simulink model "tp_thyr_rect_sm"  (R2026a)
settings: Solver=daessc  StopTime=simlength  FixedStep=Ts  MaxStep=Ts  RelTol=Ts  AbsTol=Ts  EnableMultiTasking=on
values from neighbouring files (symbols this model uses):
  I_FS = Iout_dc_nom * margin_factor    (= 103.5)    [init_model.m]
  kgrid = 1    [init_model.m]
  LFu_dc = 1.2e-3    (= 0.0012)    [init_model.m]
  pll_i1 = 80    [init_model.m]
  pll_p = 1    [init_model.m]
  RLFu_dc = 2e-4    (= 0.0002)    [init_model.m]
  Rload = 1.2/4    (= 0.3)    [init_model.m]
  Tc = 1e-5    (= 1e-05)    [init_model.m]
  Tcontrol_rect = tPWM_RECT    (= 0.0002)    [init_model.m]
  Ts = Tc/1    (= 1e-05)    [init_model.m]
  V_FS = Vout_dc_nom * margin_factor    (= 391)    [init_model.m]
  Vnom_ac_adc = 400/sqrt(3)*sqrt(2)    [init_model.m]
  Vphase1 = Vline1/sqrt(3)    [init_model.m]
  w_grid = f_grid*2*pi    (= 314.159265359)    [init_model.m]
undefined symbols (not defined in the file or in its folder): magnitude
libraries: fl_lib x248, nesl_utility x39, ee_lib x28
(part 5 of 5)

== system tp_thyr_rect_sm/Line/BR1/firing4/oscillator ==
  Data Type Conversion : DataTypeConversion  OutDataTypeStr=double  SaturateOnIntegerOverflow=off  RndMeth=Floor
  Logical Operator1 : Logic  Operator=NOT  AllPortsSameDT=off  OutDataTypeStr=boolean
  Simulink-PS Converter : nesl_utility/Simulink-PS Converter  PhysicalDomain=network_engine_domain  SubClassName=ps_input  LeftPortType=input  RightPortType=output  PseudoPeriodic=off  Frequencies=[]  NoiseDistribution=none  NoiseParameters=[]  Unit=1  AffineConversion=off  FilteringAndDerivatives=provide  SimscapeFilterOrder=1  InputFilterTimeConstant=0.001  UdotUserProvided=0
  Unit Delay1 : UnitDelay  SampleTime=Tcontrol_rect
  output : PMIOPort  Side=Right
  wires:
  Data Type Conversion/1 -> Simulink-PS Converter/1
  Unit Delay1/1 -> Logical Operator1/1
  Logical Operator1/1 -> Unit Delay1/1, Data Type Conversion/1
  connections:
  Simulink-PS Converter/RConn1 -- output/RConn1

== system tp_thyr_rect_sm/Line/BR1/firing5/oscillator ==
  Data Type Conversion : DataTypeConversion  OutDataTypeStr=double  SaturateOnIntegerOverflow=off  RndMeth=Floor
  Logical Operator1 : Logic  Operator=NOT  AllPortsSameDT=off  OutDataTypeStr=boolean
  Simulink-PS Converter : nesl_utility/Simulink-PS Converter  PhysicalDomain=network_engine_domain  SubClassName=ps_input  LeftPortType=input  RightPortType=output  PseudoPeriodic=off  Frequencies=[]  NoiseDistribution=none  NoiseParameters=[]  Unit=1  AffineConversion=off  FilteringAndDerivatives=provide  SimscapeFilterOrder=1  InputFilterTimeConstant=0.001  UdotUserProvided=0
  Unit Delay1 : UnitDelay  SampleTime=Tcontrol_rect
  output : PMIOPort  Side=Right
  wires:
  Logical Operator1/1 -> Data Type Conversion/1, Unit Delay1/1
  Unit Delay1/1 -> Logical Operator1/1
  Data Type Conversion/1 -> Simulink-PS Converter/1
  connections:
  Simulink-PS Converter/RConn1 -- output/RConn1

== system tp_thyr_rect_sm/Line/BR1/firing6/oscillator ==
  Data Type Conversion : DataTypeConversion  OutDataTypeStr=double  SaturateOnIntegerOverflow=off  RndMeth=Floor
  Logical Operator1 : Logic  Operator=NOT  AllPortsSameDT=off  OutDataTypeStr=boolean
  Simulink-PS Converter : nesl_utility/Simulink-PS Converter  PhysicalDomain=network_engine_domain  SubClassName=ps_input  LeftPortType=input  RightPortType=output  PseudoPeriodic=off  Frequencies=[]  NoiseDistribution=none  NoiseParameters=[]  Unit=1  AffineConversion=off  FilteringAndDerivatives=provide  SimscapeFilterOrder=1  InputFilterTimeConstant=0.001  UdotUserProvided=0
  Unit Delay1 : UnitDelay  SampleTime=Tcontrol_rect
  output : PMIOPort  Side=Right
  wires:
  Data Type Conversion/1 -> Simulink-PS Converter/1
  Unit Delay1/1 -> Logical Operator1/1
  Logical Operator1/1 -> Unit Delay1/1, Data Type Conversion/1
  connections:
  Simulink-PS Converter/RConn1 -- output/RConn1

== system tp_thyr_rect_sm/Line/BR2/firing1/oscillator ==
  Data Type Conversion : DataTypeConversion  OutDataTypeStr=double  SaturateOnIntegerOverflow=off  RndMeth=Floor
  Logical Operator1 : Logic  Operator=NOT  AllPortsSameDT=off  OutDataTypeStr=boolean
  Simulink-PS Converter : nesl_utility/Simulink-PS Converter  PhysicalDomain=network_engine_domain  SubClassName=ps_input  LeftPortType=input  RightPortType=output  PseudoPeriodic=off  Frequencies=[]  NoiseDistribution=none  NoiseParameters=[]  Unit=1  AffineConversion=off  FilteringAndDerivatives=provide  SimscapeFilterOrder=1  InputFilterTimeConstant=0.001  UdotUserProvided=0
  Unit Delay1 : UnitDelay  SampleTime=Tcontrol_rect
  output : PMIOPort  Side=Right
  wires:
  Data Type Conversion/1 -> Simulink-PS Converter/1
  Unit Delay1/1 -> Logical Operator1/1
  Logical Operator1/1 -> Unit Delay1/1, Data Type Conversion/1
  connections:
  Simulink-PS Converter/RConn1 -- output/RConn1

== system tp_thyr_rect_sm/Line/BR2/firing2/oscillator ==
  Data Type Conversion : DataTypeConversion  OutDataTypeStr=double  SaturateOnIntegerOverflow=off  RndMeth=Floor
  Logical Operator1 : Logic  Operator=NOT  AllPortsSameDT=off  OutDataTypeStr=boolean
  Simulink-PS Converter : nesl_utility/Simulink-PS Converter  PhysicalDomain=network_engine_domain  SubClassName=ps_input  LeftPortType=input  RightPortType=output  PseudoPeriodic=off  Frequencies=[]  NoiseDistribution=none  NoiseParameters=[]  Unit=1  AffineConversion=off  FilteringAndDerivatives=provide  SimscapeFilterOrder=1  InputFilterTimeConstant=0.001  UdotUserProvided=0
  Unit Delay1 : UnitDelay  SampleTime=Tcontrol_rect
  output : PMIOPort  Side=Right
  wires:
  Logical Operator1/1 -> Data Type Conversion/1, Unit Delay1/1
  Unit Delay1/1 -> Logical Operator1/1
  Data Type Conversion/1 -> Simulink-PS Converter/1
  connections:
  Simulink-PS Converter/RConn1 -- output/RConn1

== system tp_thyr_rect_sm/Line/BR2/firing3/oscillator ==
  Data Type Conversion : DataTypeConversion  OutDataTypeStr=double  SaturateOnIntegerOverflow=off  RndMeth=Floor
  Logical Operator1 : Logic  Operator=NOT  AllPortsSameDT=off  OutDataTypeStr=boolean
  Simulink-PS Converter : nesl_utility/Simulink-PS Converter  PhysicalDomain=network_engine_domain  SubClassName=ps_input  LeftPortType=input  RightPortType=output  PseudoPeriodic=off  Frequencies=[]  NoiseDistribution=none  NoiseParameters=[]  Unit=1  AffineConversion=off  FilteringAndDerivatives=provide  SimscapeFilterOrder=1  InputFilterTimeConstant=0.001  UdotUserProvided=0
  Unit Delay1 : UnitDelay  SampleTime=Tcontrol_rect
  output : PMIOPort  Side=Right
  wires:
  Data Type Conversion/1 -> Simulink-PS Converter/1
  Unit Delay1/1 -> Logical Operator1/1
  Logical Operator1/1 -> Unit Delay1/1, Data Type Conversion/1
  connections:
  Simulink-PS Converter/RConn1 -- output/RConn1

== system tp_thyr_rect_sm/Line/BR2/firing4/oscillator ==
  Data Type Conversion : DataTypeConversion  OutDataTypeStr=double  SaturateOnIntegerOverflow=off  RndMeth=Floor
  Logical Operator1 : Logic  Operator=NOT  AllPortsSameDT=off  OutDataTypeStr=boolean
  Simulink-PS Converter : nesl_utility/Simulink-PS Converter  PhysicalDomain=network_engine_domain  SubClassName=ps_input  LeftPortType=input  RightPortType=output  PseudoPeriodic=off  Frequencies=[]  NoiseDistribution=none  NoiseParameters=[]  Unit=1  AffineConversion=off  FilteringAndDerivatives=provide  SimscapeFilterOrder=1  InputFilterTimeConstant=0.001  UdotUserProvided=0
  Unit Delay1 : UnitDelay  SampleTime=Tcontrol_rect
  output : PMIOPort  Side=Right
  wires:
  Logical Operator1/1 -> Data Type Conversion/1, Unit Delay1/1
  Unit Delay1/1 -> Logical Operator1/1
  Data Type Conversion/1 -> Simulink-PS Converter/1
  connections:
  Simulink-PS Converter/RConn1 -- output/RConn1

== system tp_thyr_rect_sm/Line/BR2/firing5/oscillator ==
  Data Type Conversion : DataTypeConversion  OutDataTypeStr=double  SaturateOnIntegerOverflow=off  RndMeth=Floor
  Logical Operator1 : Logic  Operator=NOT  AllPortsSameDT=off  OutDataTypeStr=boolean
  Simulink-PS Converter : nesl_utility/Simulink-PS Converter  PhysicalDomain=network_engine_domain  SubClassName=ps_input  LeftPortType=input  RightPortType=output  PseudoPeriodic=off  Frequencies=[]  NoiseDistribution=none  NoiseParameters=[]  Unit=1  AffineConversion=off  FilteringAndDerivatives=provide  SimscapeFilterOrder=1  InputFilterTimeConstant=0.001  UdotUserProvided=0
  Unit Delay1 : UnitDelay  SampleTime=Tcontrol_rect
  output : PMIOPort  Side=Right
  wires:
  Data Type Conversion/1 -> Simulink-PS Converter/1
  Unit Delay1/1 -> Logical Operator1/1
  Logical Operator1/1 -> Unit Delay1/1, Data Type Conversion/1
  connections:
  Simulink-PS Converter/RConn1 -- output/RConn1

== system tp_thyr_rect_sm/Line/BR2/firing6/oscillator ==
  Data Type Conversion : DataTypeConversion  OutDataTypeStr=double  SaturateOnIntegerOverflow=off  RndMeth=Floor
  Logical Operator1 : Logic  Operator=NOT  AllPortsSameDT=off  OutDataTypeStr=boolean
  Simulink-PS Converter : nesl_utility/Simulink-PS Converter  PhysicalDomain=network_engine_domain  SubClassName=ps_input  LeftPortType=input  RightPortType=output  PseudoPeriodic=off  Frequencies=[]  NoiseDistribution=none  NoiseParameters=[]  Unit=1  AffineConversion=off  FilteringAndDerivatives=provide  SimscapeFilterOrder=1  InputFilterTimeConstant=0.001  UdotUserProvided=0
  Unit Delay1 : UnitDelay  SampleTime=Tcontrol_rect
  output : PMIOPort  Side=Right
  wires:
  Logical Operator1/1 -> Data Type Conversion/1, Unit Delay1/1
  Unit Delay1/1 -> Logical Operator1/1
  Data Type Conversion/1 -> Simulink-PS Converter/1
  connections:
  Simulink-PS Converter/RConn1 -- output/RConn1

== system tp_thyr_rect_sm/Line/C-caller ctrl/Subsystem2/oscillator ==
  In1 : Inport
  Logical Operator1 : Logic  Operator=NOT  AllPortsSameDT=off  OutDataTypeStr=boolean
  Product : Product
  Unit Delay1 : UnitDelay  SampleTime=Tcontrol_rect
  Out1 : Outport
  wires:
  Unit Delay1/1 -> Logical Operator1/1
  Logical Operator1/1 -> Product/1, Unit Delay1/1
  Product/1 -> Out1/1
  In1/1 -> Product/2

== system tp_thyr_rect_sm/Line/C-caller ctrl/Subsystem2/oscillator1 ==
  In1 : Inport
  Logical Operator1 : Logic  Operator=NOT  AllPortsSameDT=off  OutDataTypeStr=boolean
  Product : Product
  Unit Delay1 : UnitDelay  SampleTime=Tcontrol_rect
  Out1 : Outport
  wires:
  In1/1 -> Product/2
  Product/1 -> Out1/1
  Logical Operator1/1 -> Unit Delay1/1, Product/1
  Unit Delay1/1 -> Logical Operator1/1

== system tp_thyr_rect_sm/Line/C-caller ctrl/Subsystem2/oscillator2 ==
  In1 : Inport
  Logical Operator1 : Logic  Operator=NOT  AllPortsSameDT=off  OutDataTypeStr=boolean
  Product : Product
  Unit Delay1 : UnitDelay  SampleTime=Tcontrol_rect
  Out1 : Outport
  wires:
  Unit Delay1/1 -> Logical Operator1/1
  Logical Operator1/1 -> Product/1, Unit Delay1/1
  Product/1 -> Out1/1
  In1/1 -> Product/2

== system tp_thyr_rect_sm/Line/C-caller ctrl/Subsystem2/oscillator3 ==
  In1 : Inport
  Logical Operator1 : Logic  Operator=NOT  AllPortsSameDT=off  OutDataTypeStr=boolean
  Product : Product
  Unit Delay1 : UnitDelay  SampleTime=Tcontrol_rect
  Out1 : Outport
  wires:
  In1/1 -> Product/2
  Product/1 -> Out1/1
  Logical Operator1/1 -> Unit Delay1/1, Product/1
  Unit Delay1/1 -> Logical Operator1/1

== system tp_thyr_rect_sm/Line/C-caller ctrl/Subsystem2/oscillator4 ==
  In1 : Inport
  Logical Operator1 : Logic  Operator=NOT  AllPortsSameDT=off  OutDataTypeStr=boolean
  Product : Product
  Unit Delay1 : UnitDelay  SampleTime=Tcontrol_rect
  Out1 : Outport
  wires:
  Unit Delay1/1 -> Logical Operator1/1
  Logical Operator1/1 -> Product/1, Unit Delay1/1
  Product/1 -> Out1/1
  In1/1 -> Product/2

== system tp_thyr_rect_sm/Line/C-caller ctrl/Subsystem2/oscillator5 ==
  In1 : Inport
  Logical Operator1 : Logic  Operator=NOT  AllPortsSameDT=off  OutDataTypeStr=boolean
  Product : Product
  Unit Delay1 : UnitDelay  SampleTime=Tcontrol_rect
  Out1 : Outport
  wires:
  In1/1 -> Product/2
  Product/1 -> Out1/1
  Logical Operator1/1 -> Unit Delay1/1, Product/1
  Unit Delay1/1 -> Logical Operator1/1

== system tp_thyr_rect_sm/Line/phase_gen/pll_stageA/abc2alphabeta ==
  Vgrid_ab : Inport
  Vgrid_bc : Inport  Port=2
  Vgrid_ca : Inport  Port=3
  Gain : Gain
  Gain7 : Gain  Gain=-1
  Zero-Order Hold : ZeroOrderHold  SampleTime=Tcontrol_rect
  Zero-Order Hold1 : ZeroOrderHold  SampleTime=Tcontrol_rect
  Zero-Order Hold2 : ZeroOrderHold  SampleTime=Tcontrol_rect
  abc2alphabeta : Subsystem
  Vgrid_alpha : Outport
  Vgrid_beta : Outport  Port=2
  wires:
  Vgrid_ab/1 -> Zero-Order Hold/1
  Vgrid_bc/1 -> Zero-Order Hold1/1
  Vgrid_ca/1 -> Zero-Order Hold2/1
  Zero-Order Hold/1 -> abc2alphabeta/1(a)
  Zero-Order Hold1/1 -> abc2alphabeta/2(b)
  Zero-Order Hold2/1 -> abc2alphabeta/3(c)
  abc2alphabeta/2("beta ") -> Gain7/1
  abc2alphabeta/1("alpha ") -> Gain/1
  Gain/1 -> Vgrid_beta/1
  Gain7/1 -> Vgrid_alpha/1

== system tp_thyr_rect_sm/Line/phase_gen/pll_stageB/alphabeta2xieta ==
  alpha : Inport
  beta : Inport  Port=2
  wt : Inport  Port=3
  Product{,1..3} (4 alike) : Product  RndMeth=Zero
  Sum : Sum
  Sum1 : Sum  Inputs=-+
  Trigonometric Function : Trigonometry  Operator=cos
  Trigonometric Function1 : Trigonometry
  xi : Outport
  eta : Outport  Port=2
  wires:
  Trigonometric Function/1 -> [cos]
  Trigonometric Function1/1 -> [sin]
  wt/1 -> Trigonometric Function1/1, Trigonometric Function/1
  Sum1/1 -> eta/1
  Sum/1 -> xi/1
  [cos] -> Product3/1
  Product3/1 -> Sum1/2
  Product2/1 -> Sum1/1
  [sin] -> Product2/1
  beta/1 -> Product3/2, Product1/2
  [sin] -> Product1/1
  Product1/1 -> Sum/2
  Product/1 -> Sum/1
  alpha/1 -> Product2/2, Product/2
  [cos] -> Product/1

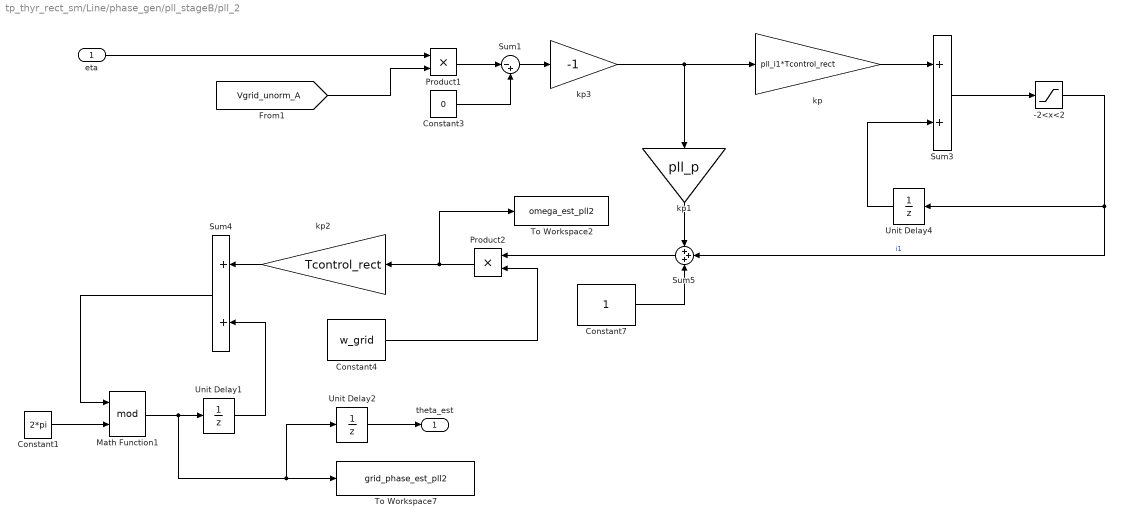
== system tp_thyr_rect_sm/Line/phase_gen/pll_stageB/pll_2 ==
  eta : Inport
  -2<x<2 : Saturate  UpperLimit=2  LowerLimit=-2
  Constant1 : Constant  Value=2*pi
  Constant3 : Constant  Value=0
  Constant4 : Constant  Value=w_grid
  Constant7 : Constant
  Math Function1 : Math  Operator=mod  SignedPower=on
  Product1 : Product  RndMeth=Zero
  Product2 : Product  RndMeth=Zero
  Sum1 : Sum  Inputs=|-+
  Sum3 : Sum  SaturateOnIntegerOverflow=on
  Sum4 : Sum  SaturateOnIntegerOverflow=on
  Sum5 : Sum  Inputs=+++
  To Workspace2 : ToWorkspace  VariableName=omega_est_pll2  SampleTime=Tc
      settings: MaxDataPoints=Nc
  To Workspace7 : ToWorkspace  VariableName=grid_phase_est_pll2  SampleTime=Tc
      settings: MaxDataPoints=Nc
  Unit Delay1 : UnitDelay  SampleTime=Tcontrol_rect
  Unit Delay2 : UnitDelay  SampleTime=Tcontrol_rect
  Unit Delay4 : UnitDelay  SampleTime=Tcontrol_rect
  kp : Gain  Gain=pll_i1*Tcontrol_rect  SaturateOnIntegerOverflow=on  OutDataTypeStr=Inherit: Same as input  ParamDataTypeStr=Inherit: Same as input
  kp1 : Gain  Gain=pll_p  SaturateOnIntegerOverflow=on  OutDataTypeStr=Inherit: Same as input  ParamDataTypeStr=Inherit: Same as input
  kp2 : Gain  Gain=Tcontrol_rect  SaturateOnIntegerOverflow=on  OutDataTypeStr=Inherit: Same as input  ParamDataTypeStr=Inherit: Same as input
  kp3 : Gain  Gain=-1  SaturateOnIntegerOverflow=on  OutDataTypeStr=Inherit: Same as input  ParamDataTypeStr=Inherit: Same as input
  theta_est : Outport
  wires:
  Constant7/1 -> Sum5/3
  Constant3/1 -> Sum1/2
  [Vgrid_unorm_A] -> Product1/2
  Product2/1 -> kp2/1, To Workspace2/1
  kp/1 -> Sum3/1
  Sum4/1 -> Math Function1/1
  kp1/1 -> Sum5/1
  Product1/1 -> Sum1/1
  Sum1/1 -> kp3/1
  Unit Delay2/1 -> theta_est/1
  -2<x<2/1 -> Unit Delay4/1, Sum5/2  "i1"
  Unit Delay4/1 -> Sum3/2
  Sum3/1 -> -2<x<2/1
  kp2/1 -> Sum4/1
  Sum5/1 -> Product2/1
  Constant4/1 -> Product2/2
  Unit Delay1/1 -> Sum4/2
  Math Function1/1 -> Unit Delay2/1, To Workspace7/1, Unit Delay1/1
  Constant1/1 -> Math Function1/2
  eta/1 -> Product1/1
  kp3/1 -> kp/1, kp1/1

== system tp_thyr_rect_sm/Line/phase_gen/pll_stageA/abc2alphabeta/abc2alphabeta ==
  a : Inport
  b : Inport  Port=2
  c : Inport  Port=3
  Gain1 : Gain  Gain=-1/2
  Gain11 : Gain  Gain=-1/2
  Gain2 : Gain  Gain=0
  Gain3 : Gain  Gain=-sqrt(3)/2
  Gain4 : Gain  Gain=sqrt(3)/2
  Gain8 : Gain  Gain=2/3
  Gain9 : Gain  Gain=2/3
  Sum : Sum  Inputs=+++
  Sum1 : Sum  Inputs=+++
  "alpha " : Outport
  "beta " : Outport  Port=2
  wires:
  Sum1/1 -> Gain9/1
  Sum/1 -> Gain8/1
  Gain4/1 -> Sum/2
  Gain2/1 -> Sum/1
  a/1 -> Gain2/1, Sum1/1
  Gain3/1 -> Sum/3
  b/1 -> Gain4/1, Gain11/1
  c/1 -> Gain3/1, Gain1/1
  Gain1/1 -> Sum1/3
  Gain11/1 -> Sum1/2
  Gain9/1 -> "alpha "/1
  Gain8/1 -> "beta "/1

== matlab function tp_thyr_rect_sm/Line/C-caller ctrl/MATLAB Function ==
  data: theta input; pulses output; alpha input; pulse_width_deg input
function pulses = thyristor_firing_12p(theta, alpha, pulse_width_deg)
% THYRISTOR_FIRING_12P - Generatore firing 12 impulsi per ponte Yyd
%
% Ingressi:
%   theta          : fase istantanea [0, 2*pi] (rad)
%   alpha          : angolo di ritardo di accensione (rad)
%   pulse_width_deg: durata impulso in gradi (default 110)
%
% Uscita:
%   pulses : vettore [12x1] logico, impulso attivo = 1
%
% Ponte 12 impulsi Yyd:
%   - Ponte superiore (Y/Y): thyristori T1..T6, sfasati 60 deg
%   - Ponte inferiore (Y/D): thyristori T7..T12, sfasati 60 deg + 30 deg offset
%
% Angoli naturali di commutazione (fase A come riferimento):
%   Ponte Y/Y:  30, 90, 150, 210, 270, 330 deg  (pi/6 + k*pi/3)
%   Ponte Y/D:  60, 120, 180, 240, 300, 360 deg  (pi/3 + k*pi/3, ovvero +30 deg)

if nargin < 3 || isempty(pulse_width_deg)
    pulse_width_deg = 110;
end

pw = pulse_width_deg * pi / 180;  % durata impulso in radianti

% --- Angoli naturali di commutazione (rad) ---
% Ponte Y/Y (6 thyristori): sfasati 60 deg partendo da 30 deg
natural_YY = pi/6 + (0:5)' * (pi/3);   % [6x1]

% Ponte Y/D (6 thyristori): offset di +30 deg rispetto a Y/Y
natural_YD = natural_YY + pi/6;         % [6x1]

% Angoli di firing con ritardo alpha
firing_YY = natural_YY + alpha;  % [6x1]
firing_YD = natural_YD + alpha;  % [6x1]

% Tutti i 12 angoli di firing (T1..T6 = YY, T7..T12 = YD)
firing_all = [firing_YY; firing_YD];  % [12x1]

% Normalizzare theta in [0, 2*pi)
theta_norm = mod(theta, 2*pi);

% --- Calcolo impulsi ---
% Impulso attivo se: theta_norm in [firing_i, firing_i + pw] (mod 2*pi)
pulses = false(12, 1);

for k = 1:12
    f = mod(firing_all(k), 2*pi);      % angolo firing normalizzato
    f_end = mod(f + pw, 2*pi);         % fine impulso normalizzato
    
    if f_end > f
        % Caso normale: nessun wrap-around
        pulses(k) = (theta_norm >= f) && (theta_norm < f_end);
    else
        % Caso wrap-around (l'impulso supera 2*pi)
        pulses(k) = (theta_norm >= f) || (theta_norm < f_end);
    end
end

end
